simulink model "Lab2_Task_2_mstraj"  (R2025b)
settings: Solver=FixedStepAuto  StartTime=0.0  StopTime=inf  RelTol=1e-3
model workspace (MAT data in the model file):
  SL_ROS_VariableLengthArrays_MaxSizes.CommonInfo.ArrayTruncateAction = 'EmitWarning'
  SL_ROS_VariableLengthArrays_MaxSizes.MsgTypeMap = containers.Map
  SL_ROS_VariableLengthArrays_MaxSizes.MsgTypeMap.serialization.keys = {'sensor_msgs/LaserScan'}
  SL_ROS_VariableLengthArrays_MaxSizes.MsgTypeMap.serialization.values{1}(1).PropertyName = 'intensities'
  SL_ROS_VariableLengthArrays_MaxSizes.MsgTypeMap.serialization.values{1}(1).DataType = 'single'
  SL_ROS_VariableLengthArrays_MaxSizes.MsgTypeMap.serialization.values{1}(1).MaxLength = 360
  SL_ROS_VariableLengthArrays_MaxSizes.MsgTypeMap.serialization.values{1}(2).PropertyName = 'ranges'
  SL_ROS_VariableLengthArrays_MaxSizes.MsgTypeMap.serialization.values{1}(2).DataType = 'single'
  SL_ROS_VariableLengthArrays_MaxSizes.MsgTypeMap.serialization.values{1}(2).MaxLength = 360
  SL_ROS_VariableLengthArrays_MaxSizes.MsgTypeMap.serialization.uniformity = 0
  SL_ROS_VariableLengthArrays_MaxSizes.MsgTypeMap.serialization.keyType = 'char'
  SL_ROS_VariableLengthArrays_MaxSizes.MsgTypeMap.serialization.valueType = 'any'
undefined symbols (not defined in the file or in its folder): header, traj_Sinusoidal, traj_Six, traj_square, twist
libraries: ros2lib x4
settings Model: Creator=scott  LastModifiedBy=abodynasser22
settings OptimizationCC: DefaultParameterBehavior=Inlined  EnhancedBackFolding=on  PassReuseOutputArgsAs=Individual arguments  ZeroExternalMemoryAtStartup=off  ZeroInternalMemoryAtStartup=off  MaxStackSize=64  OptimizeBlockOrder=speed  DifferentSizesBufferReuse=on  OptimizationCustomize=off  EfficientTunableParamExpr=on
settings DebuggingCC: ParameterTunabilityLossMsg=error
settings HardwareCC: ProdBitPerPointer=32.0  ProdBitPerSizeT=32.0  ProdBitPerPtrDiffT=32.0  ProdWordSize=32.0  ProdHWDeviceType=Intel->x86-32 (Windows32)  UseEmbeddedCoderFeatures=off
settings SFSimCC: MATLABDynamicMemAlloc=off
settings RTWCC: SystemTargetFile=ert.tlc  HardwareBoard=Robot Operating System 2 (ROS 2)  TLCOptions="-aInlineSetEventsForThisBaseRateFcn=TLC_FALSE -aSuppressMultiTaskScheduler=TLC_FALSE  -aRateBasedStepFcn=0"  TemplateMakefile=ert_default_tmf  Toolchain=Colcon Tools  TargetLang=C++  Description=Embedded Coder
settings CodeAppCC: ForceParamTrailComments=on  IgnoreCustomStorageClasses=off  OperatorAnnotations=on  SimulinkDataObjDesc=on  SFDataObjDesc=on  InsertBlockDesc=on
settings ERTTargetCC: ExtModeTransport=2.0  ExtModeStaticAlloc=on  ExtModeAutomaticAllocSize=off  ExtModeMexFile=ext_xcp  ExtModeIntrfLevel=Level2 - Open  RootIOFormat=Structure reference  CodeInterfacePackaging=C++ class  SupportNonInlinedSFcns=on

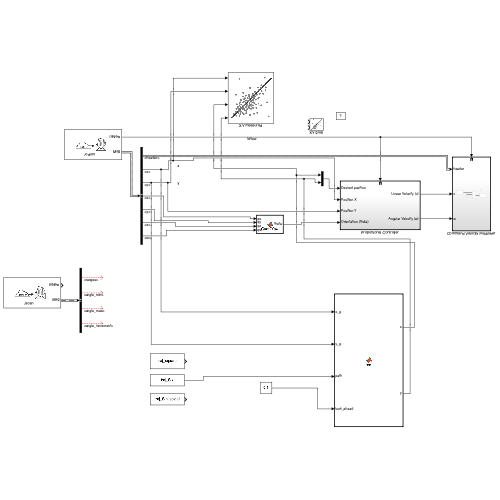
[thumbnail: Simulink's stored preview of the top-level diagram]
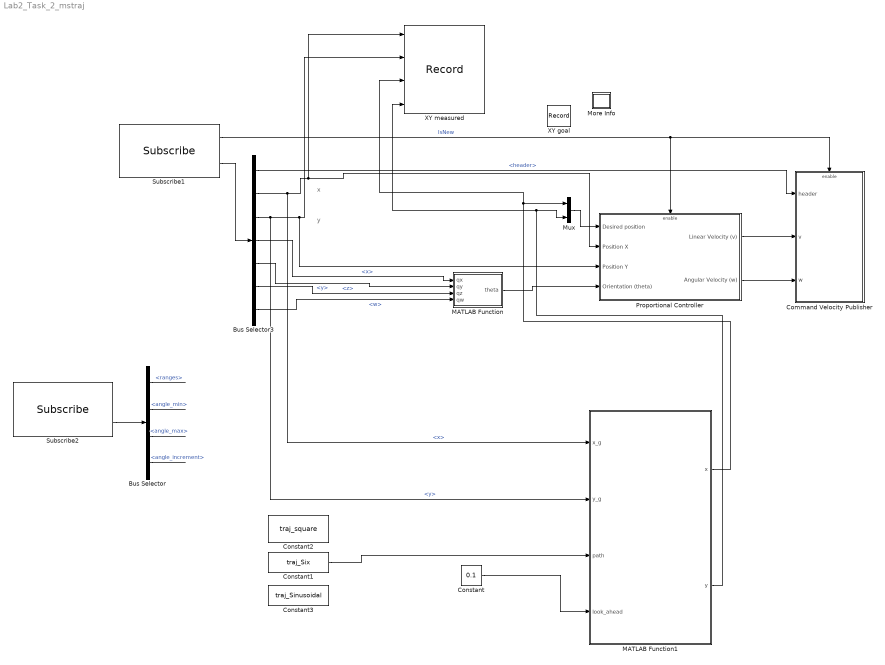
== system Lab2_Task_2_mstraj ==
  note: y
  note: x
  Bus Selector : BusSelector  OutputSignals=ranges,angle_min,angle_max,angle_increment
  Bus Selector3 : BusSelector  OutputSignals=header,pose.pose.position.x,pose.pose.position.y,pose.pose.orientation.x,pose.pose.orientation.y,pose.pose.orientation.z,pose.pose.orientation.w
  Command Velocity Publisher : Subsystem
  Constant : Constant  Value=0.1
  Constant1 : Constant  Value=traj_Six
  Constant2 : Constant  Value=traj_square
  Constant3 : Constant  Value=traj_Sinusoidal
  MATLAB Function : MATLAB Function  TreatAsAtomicUnit=on
  MATLAB Function1 : MATLAB Function  TreatAsAtomicUnit=on
  More Info : Subsystem
      settings: OpenFcn=showdemo(bdroot(gcb))
      mask Display: disp('?')
  Mux : Mux  Inputs=2
  Proportional Controller : Subsystem
  Subscribe1 : ros2lib/Subscribe  topicSource=Select from ROS network  topic=/odom  messageType=nav_msgs/Odometry  sampleTime=-1  QOSHistory=Keep last  QOSDepth=10  QOSReliability=Reliable  QOSDurability=Volatile  QOSDeadline=Inf  QOSLifespan=Inf  QOSLiveliness=Automatic  QOSLeaseDuration=Inf  QOSAvoidROSNamespaceConventions=off
  Subscribe2 : ros2lib/Subscribe  topicSource=Select from ROS network  topic=/scan  messageType=sensor_msgs/LaserScan  sampleTime=-1  QOSHistory=Keep last  QOSDepth=10  QOSReliability=Best effort  QOSDurability=Volatile  QOSDeadline=Inf  QOSLifespan=Inf  QOSLiveliness=Automatic  QOSLeaseDuration=Inf  QOSAvoidROSNamespaceConventions=off
  XY goal : Record  NumPorts=2.0  FileSettingsInternal="{\"entries\":[{\"content\":{\"excelSettings\":{\"content\":{},\"type\":\"Streamout.ExcelSettings\"},\"parquetSettings\":{\"content\":{},\"type\":\"Streamout.ParquetSettings\"}},\"type\":\"Streamout.FileSettingStorage\",\"uuid\":\"\"}],\"packageUris\":[\"http:\\/\\/schema.mathworks.com\\/mf0\\/streamout_blocks\\/R2020a\"],\"version\":\"1.0\"}"  FrameSettings=[0, 0]  Layout=[1 1]  SignalsInternal="{\"entries\":[{\"content\":{\"signals\":[{\"content\":{\"blockPath\":[],\"dimensions\":[1],\"domain\":\"\",\"lineColor\":\"#fe330a\",\"lineWidth\":2,\"plots\":[ 1 ],\"port\":1,\"sid\":[\"\"],\"signalID\":1},\"type\":\"RecordBlkView.Signal\",\"uuid\":\"\"},{\"content\":{\"blockPath\":[],\"dimensions\":[1],\"domain\":\"\",\"lineColor\":\"#22b573\",\"lineWidth\":2,\"plots\":[ 1 ],\"port\":2,\"sid\":[\"\"],\"signalID\":2},\"type\":\"RecordBlkView.Signal\",\"uuid\":\"\"}]},\"type\":\"RecordBlkView.InputSignals\",\"uuid\":\"\"}],\"packageUris\":[\"http:\\/\\/schema.mathworks.com\\/mf0\\/streamout_blocks\\/R2020a\"],\"version\":\"1.0\"}"  VisualizationBindings="{\"xyplotplugin\":{\"info\":[{\"series\":[{\"bindingParametersList\":[{\"parameter\":\"X-Axis\",\"signalID\":1,\"signalName\":\"XY goal:1\"},{\"parameter\":\"Y-Axis\",\"signalID\":2,\"signalName\":\"XY goal:2\"}],\"seriesID\":0}],\"subplotID\":1}]}}"  CompatibilityTag=XY
  XY measured : Record  NumPorts=4.0  FileSettingsInternal="{\"entries\":[{\"content\":{\"excelSettings\":{\"content\":{},\"type\":\"Streamout.ExcelSettings\"},\"parquetSettings\":{\"content\":{},\"type\":\"Streamout.ParquetSettings\"}},\"type\":\"Streamout.FileSettingStorage\",\"uuid\":\"\"}],\"packageUris\":[\"http:\\/\\/schema.mathworks.com\\/mf0\\/streamout_blocks\\/R2020a\"],\"version\":\"1.0\"}"  FrameSettings=[0, 0, 0, 0]  Layout=[1 1]  SignalsInternal="{\"entries\":[{\"content\":{\"signals\":[{\"content\":{\"blockPath\":[],\"dimensions\":[1],\"domain\":\"\",\"lineColor\":\"#0072bd\",\"lineWidth\":2,\"plots\":[ 1 ],\"port\":1,\"sid\":[\"\"],\"signalID\":1,\"signalName\":\"<x>\"},\"type\":\"RecordBlkView.Signal\",\"uuid\":\"\"},{\"content\":{\"blockPath\":[],\"dimensions\":[1],\"domain\":\"\",\"lineColor\":\"#0072bd\",\"lineWidth\":2,\"plots\":[ 1 ],\"port\":2,\"sid\":[\"\"],\"signalID\":2,\"signalName\":\"<y>\"},\"type\":\"RecordBlkView.Signal\",\"uuid\":\"\"},{\"content\":{\"blockPath\":[],\"dimensions\":[1],\"domain\":\"\",\"lineColor\":\"#fe330a\",\"lineWidth\":2,\"plots\":[ 1 ],\"port\":3,\"sid\":[\"\"],\"signalID\":3,\"signalName\":\"MATLAB Function1:1\"},\"type\":\"RecordBlkView.Signal\",\"uuid\":\"\"},{\"content\":{\"blockPath\":[],\"dimensions\":[1],\"domain\":\"\",\"lineColor\":\"#fe330a\",\"lineWidth\":2,\"plots\":[ 1 ],\"port\":4,\"sid\":[\"\"],\"signalID\":4,\"signalName\":\"MATLAB Function1:2\"},\"type\":\"RecordBlkView.Signal\",\"uuid\":\"\"}]},\"type\":\"RecordBlkView.InputSignals\",\"uuid\":\"\"}],\"packageUris\":[\"http:\\/\\/schema.mathworks.com\\/mf0\\/streamout_blocks\\/R2020a\"],\"version\":\"1.0\"}"  VisualizationBindings="{\"xyplotplugin\":{\"info\":[{\"series\":[{\"bindingParametersList\":[{\"parameter\":\"X-Axis\",\"signalID\":1,\"signalName\":\"<x>\"},{\"parameter\":\"Y-Axis\",\"signalID\":2,\"signalName\":\"<y>\"},{\"parameter\":\"X-Axis\",\"signalID\":1,\"signalName\":\"<x>\"},{\"parameter\":\"Y-Axis\",\"signalID\":2,\"signalName\":\"<y>\"},{\"parameter\":\"X-Axis\",\"signalID\":1,\"signalName\":\"<x>\"},{\"parameter\":\"Y-Axis\",\"signalID\":2,\"signalName\":\"<y>\"},{\"parameter\":\"X-Axis\",\"signalID\":1,\"signalName\":\"<x>\"},{\"parameter\":\"Y-Axis\",\"signalID\":2,\"signalName\":\"<y>\"}],\"seriesID\":0},{\"bindingParametersList\":[{\"parameter\":\"X-Axis\",\"signalID\":3,\"signalName\":\"MATLAB Function1:1\"},{\"parameter\":\"Y-Axis\",\"signalID\":4,\"signalName\":\"MATLAB Function1:2\"}],\"seriesID\":1}],\"subplotID\":1}]}}"  CompatibilityTag=XY
  wires:
  Subscribe1/2 -> Bus Selector3/1
  Subscribe1/1 -> Command Velocity Publisher/Enable, Proportional Controller/Enable  "IsNew"
  Proportional Controller/1(Linear Velocity (v)) -> Command Velocity Publisher/2(v)
  Proportional Controller/2(Angular Velocity (w)) -> Command Velocity Publisher/3(w)
  Bus Selector3/1 -> Command Velocity Publisher/1(header)  "<header>"
  Bus Selector3/2 -> MATLAB Function1/1(x_g), XY measured/1, Proportional Controller/2(Position X)  "<x>"
  Bus Selector3/3 -> MATLAB Function1/2(y_g), XY measured/2, Proportional Controller/3(Position Y)  "<y>"
  Bus Selector3/4 -> MATLAB Function/1(qx)  "<x>"
  Bus Selector3/5 -> MATLAB Function/2(qy)  "<y>"
  Bus Selector3/6 -> MATLAB Function/3(qz)  "<z>"
  Bus Selector3/7 -> MATLAB Function/4(qw)  "<w>"
  Subscribe2/2 -> Bus Selector/1
  Bus Selector/1 -> ?  "<ranges>"
  Bus Selector/2 -> ?  "<angle_min>"
  Bus Selector/3 -> ?  "<angle_max>"
  Bus Selector/4 -> ?  "<angle_increment>"
  MATLAB Function/1(theta) -> Proportional Controller/4(Orientation (theta))
  Mux/1 -> Proportional Controller/1(Desired position)
  MATLAB Function1/1(x) -> XY measured/3, Mux/1
  MATLAB Function1/2(y) -> Mux/2, XY measured/4
  Constant/1 -> MATLAB Function1/4(look_ahead)
  Constant1/1 -> MATLAB Function1/3(path)

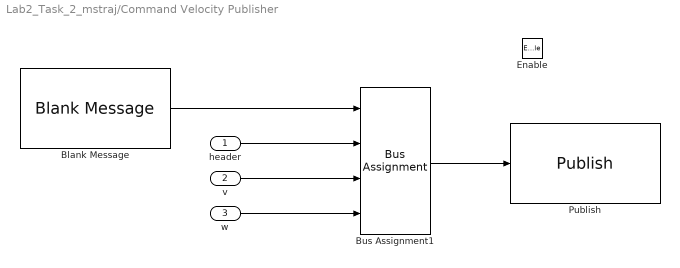
== system Lab2_Task_2_mstraj/Command Velocity Publisher ==
  header : Inport
  v : Inport  Port=2
  w : Inport  Port=3
  Enable : EnablePort
  Blank Message : ros2lib/Blank Message  messageClass=Message  entityType=geometry_msgs/TwistStamped  messageType=geometry_msgs/TwistStamped  SampleTime=inf
  Bus Assignment1 : BusAssignment  DialogController=Simulink.DDGSource_BusAssignment  AssignedSignals=header,twist.linear.x,twist.angular.z
  Publish : ros2lib/Publish  topicSource=Select from ROS network  topic=/cmd_vel  messageType=geometry_msgs/TwistStamped  QOSHistory=Keep last  QOSDepth=10  QOSReliability=Reliable  QOSDurability=Volatile  QOSDeadline=Inf  QOSLifespan=Inf  QOSLiveliness=Automatic  QOSLeaseDuration=Inf  QOSAvoidROSNamespaceConventions=off
  wires:
  Bus Assignment1/1 -> Publish/1
  Blank Message/1 -> Bus Assignment1/1
  header/1 -> Bus Assignment1/2
  v/1 -> Bus Assignment1/3
  w/1 -> Bus Assignment1/4

== system Lab2_Task_2_mstraj/More Info ==

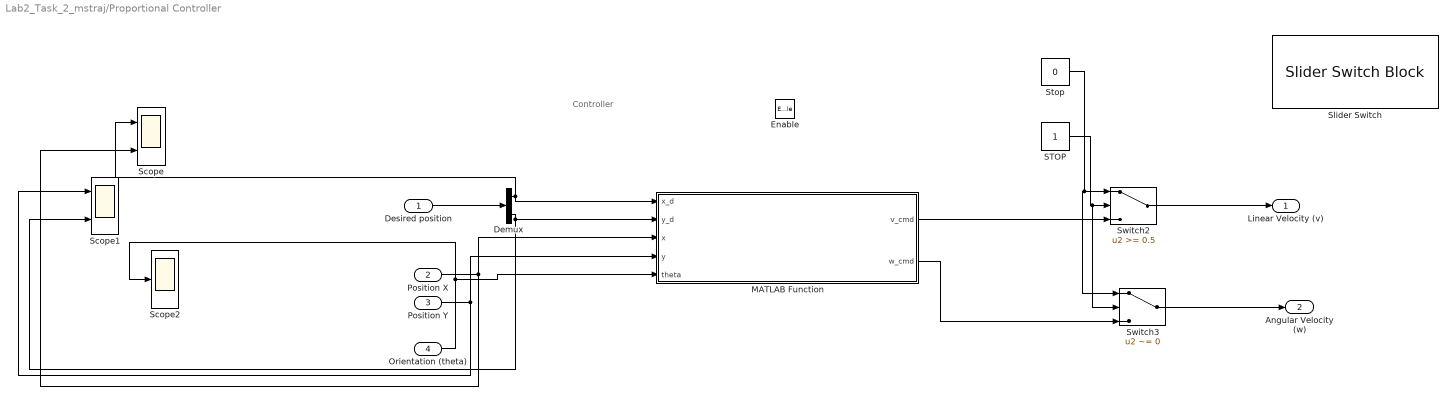
== system Lab2_Task_2_mstraj/Proportional Controller ==
  note: Controller
  Desired position : Inport
  Position X : Inport  Port=2
  Position Y : Inport  Port=3
  Orientation (theta) : Inport  Port=4
  Enable : EnablePort
  Demux : Demux  Outputs=2
  MATLAB Function : MATLAB Function  TreatAsAtomicUnit=on
  "STOP " : Constant
  Scope : Scope  NumInputPorts=2
      settings: ActiveDisplayYMinimum=-0.089125023360917932  ActiveDisplayYMaximum=0.58942881968958882
  Scope1 : Scope  NumInputPorts=2
      settings: ActiveDisplayYMinimum=-0.093278365244541847  ActiveDisplayYMaximum=0.58747839482851516  DataLoggingVariableName=ScopeData2
  Scope2 : Scope
      settings: ActiveDisplayYMinimum=-3.8970182021452358  ActiveDisplayYMaximum=3.895302128785882  DataLoggingVariableName=ScopeData3
  Slider Switch : SliderSwitchBlock
  Stop : Constant  Value=0
  Switch2 : Switch  Threshold=0.5  SaturateOnIntegerOverflow=off  InputSameDT=off
  Switch3 : Switch  Criteria=u2 ~= 0  Threshold=0.5  SaturateOnIntegerOverflow=off  InputSameDT=off
  Linear Velocity (v) : Outport  VectorParamsAs1DForOutWhenUnconnected=off
  Angular Velocity (w) : Outport  Port=2  VectorParamsAs1DForOutWhenUnconnected=off
  wires:
  Stop/1 -> Switch3/1, Switch2/1
  "STOP "/1 -> Switch3/2, Switch2/2
  Switch2/1 -> Linear Velocity (v)/1
  Switch3/1 -> Angular Velocity (w)/1
  Desired position/1 -> Demux/1
  Demux/1 -> Scope/1, MATLAB Function/1(x_d)
  Demux/2 -> Scope1/2, MATLAB Function/2(y_d)
  Position X/1 -> Scope/2, MATLAB Function/3(x)
  Orientation (theta)/1 -> Scope2/1, MATLAB Function/5(theta)
  Position Y/1 -> MATLAB Function/4(y), Scope1/1
  MATLAB Function/1(v_cmd) -> Switch2/3
  MATLAB Function/2(w_cmd) -> Switch3/3

== matlab function Lab2_Task_2_mstraj/MATLAB Function ==
  data: qx input; theta output; qy input; qz input; qw input
function theta = Quat2Yaw(qx, qy, qz, qw)
%#codegen
% Inputs are quaternion components from /odom:
% orientation.x = qx, .y = qy, .z = qz, .w = qw

% Build 1x4 quaternion row in the order [w x y z]
q = [qw, qx, qy, qz];

% Convert to Euler angles [yaw pitch roll] (ZYX convention)
eul = quat2eul(q, 'ZYX');

% Use yaw (rotation about Z-axis)
theta = eul(1);
end

== matlab function Lab2_Task_2_mstraj/Proportional Controller/MATLAB Function ==
  data: x_d input; v_cmd output; y_d input; x input; y input; theta input; w_cmd output
function [v_cmd, w_cmd] = pose_controller(x_d, y_d, x, y, theta)
%#codegen
% Enkel P-regulator för differentialdriven robot

% --- parametrar (tune vid behov) ---
Kv = 0.7;      % linjär hastighetsförstärkning
Kw = 1;      % vinkelhastighetsförstärkning
d_stop = 0.05; % stopp-radie [m]

% --- fel i position ---
dx = x_d - x;
dy = y_d - y;

% Avstånd till mål
d = sqrt(dx^2 + dy^2);

% Vinkel mot mål i världssystemet
theta_goal = atan2(dy, dx);

% Vinkelfel (wrap till [-pi, pi])
alpha = theta_goal - theta;      
alpha = atan2(sin(alpha), cos(alpha));

% --- P-lagar ---
v_cmd = Kv * d;       %Velocity (Linjär hastigher)
w_cmd = Kw * alpha;   %Angular Velocity (Vinkel hastighet)

% --- Stanna när vi är nära målet ---
if d < d_stop
    v_cmd = 0;
    w_cmd = 0;
end
end

== matlab function Lab2_Task_2_mstraj/MATLAB Function1 ==
  data: x output; x_g input; y output; y_g input; path input size=[103 2]; look_ahead input
function [x,y] = fcn(x_g, y_g, path, look_ahead)
persistent i;
if isempty(i)
    i = 1;
end
x_path = path(i, 1);
y_path = path(i, 2);
distance = sqrt((x_path - x_g)^2 + (y_path - y_g)^2);

if distance <= look_ahead %&& abs(diff) <= yaw_margin
    i = i+1;
    if i > size(path, 1)
        i = 1;
    end
end

x = path(i, 1);
y = path(i, 2);
